simulink model "BLDC_SMO"  (R2024b)
settings: Solver=ode3  StartTime=0.0  StopTime=5  FixedStep=1e-6  RelTol=1e-3
libraries: spsMosfetLib x6, spsCurrentMeasurementLib x3, spsVoltageMeasurementLib x3, simulink x2, spsDCVoltageSourceLib x1, slpidlib x1, spsPermanentMagnetSynchronousMachineLib x1, spspowerguiLib x1
settings Model: Creator=sinha  LastModifiedBy=sinha

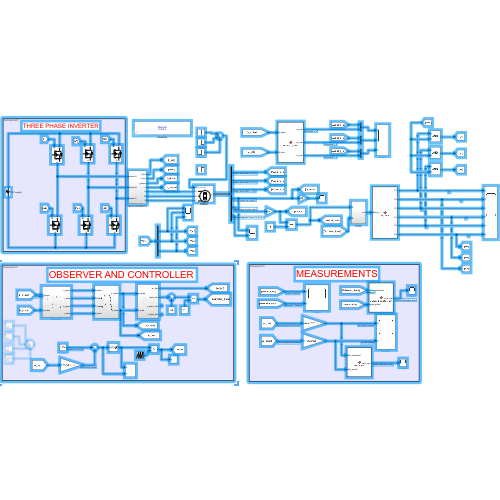
[thumbnail: Simulink's stored preview of the top-level diagram]
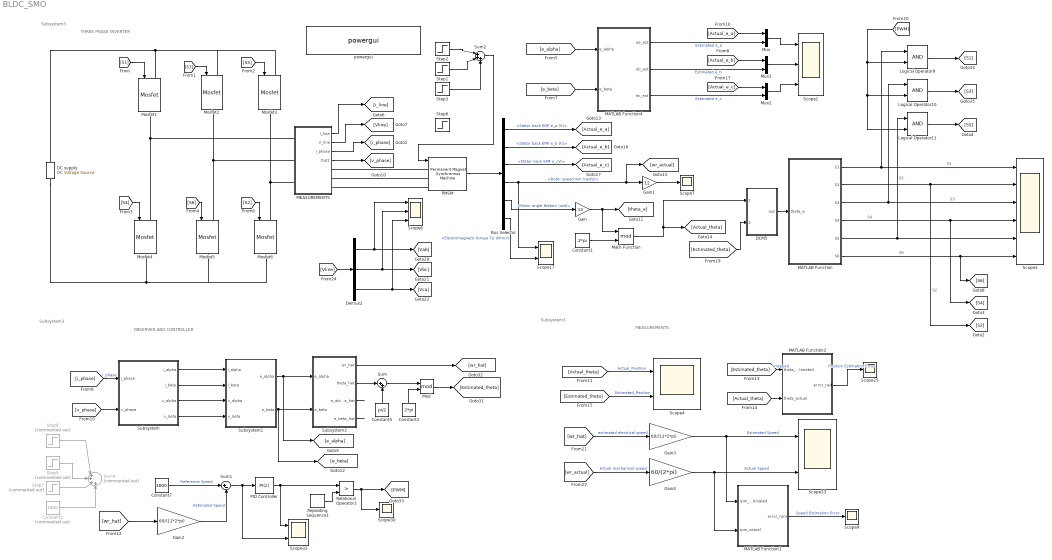
== system BLDC_SMO ==
  note: THREE PHASE INVERTER
  note: Subsystem3
  note: MEASUREMENTS
  note: OBSERVER AND CONTROLLER
  note: Subsystem3
  note: Subsystem3
  Bus Selector : BusSelector  OutputSignals=Stator back EMF e_a (V),Stator back EMF e_b (V),Stator back EMF e_cV),Rotor speed wm (rad/s),Rotor angle thetam (rad),Electromagnetic torque Te (N*m)
  Constant1 : Constant  Value=2*pi
  Constant2 : Constant  Commented=on  Value=1000
  Constant3 : Constant  Value=2*pi
  Constant5 : Constant  Value=pi/2
  Constant7 : Constant  Value=1000
  DC supply : spsDCVoltageSourceLib/DC Voltage Source  Amplitude=120  Measurements=None
  DCM5 : Subsystem
  Demux2 : Demux  Outputs=3
  Gain : Gain  Gain=12
  Gain1 : Gain  Gain=12
  Gain2 : Gain  Gain=60/(12*2*pi)
  Gain3 : Gain  Gain=60/(12*2*pi)
  Gain4 : Gain  Gain=60/(2*pi)
  Logical Operator10 : Logic  AllPortsSameDT=off  OutDataTypeStr=boolean
  Logical Operator11 : Logic  AllPortsSameDT=off  OutDataTypeStr=boolean
  Logical Operator9 : Logic  AllPortsSameDT=off  OutDataTypeStr=boolean
  MATLAB Function : MATLAB Function  TreatAsAtomicUnit=on
  MATLAB Function1 : MATLAB Function  TreatAsAtomicUnit=on  SystemSampleTime=1e-4
  MATLAB Function2 : MATLAB Function  TreatAsAtomicUnit=on  SystemSampleTime=1e-4
  MATLAB Function4 : MATLAB Function  TreatAsAtomicUnit=on  SystemSampleTime=1e-4
  MEASUREMENTS : Subsystem
  Math Function : Math  Operator=mod
  Mod : Math  Operator=mod
  Mosfet{1..6} (6 alike) : spsMosfetLib/Mosfet  Ron=0.1  Lon=0  Rd=0.01  Vfd=0  IC=0  Rs=1e5  Cs=inf  Measurements=off
  Mux : Mux  Inputs=2
  Mux1 : Mux  Inputs=2
  Mux2 : Mux  Inputs=2
  PID Controller : slpidlib/PID Controller  Controller=PI  Form=Parallel  TimeDomain=Discrete-time  UseExternalTs=off  SampleTime=1e-3  IntegratorMethod=Forward Euler  FilterMethod=Forward Euler  ControllerParametersSource=internal  P=0.01  I=0.05  UseKiTs=off  D=0  UseExternalDerivativeSource=off  N=100  UseFilter=on  TunerSelectOption=Transfer Function Based (PID Tuner App)  InitialConditionSource=internal  InitialConditionForIntegrator=0  InitialConditionForFilter=0  DifferentiatorICPrevScaledInput=0  ExternalReset=none  TrackingMode=off  Kt=1  LimitOutput=on  SatLimitsSource=internal  UpperSaturationLimit=1  LowerSaturationLimit=0  LinearizeAsGain=on  AntiWindupMode=back-calculation  Kb=1  LimitIntegrator=off  UpperIntegratorSaturationLimit=inf  LowerIntegratorSaturationLimit=-inf  POutMin=[]  POutMax=[]  IOutMin=[]  IOutMax=[]  DOutMin=[]  DOutMax=[]  NOutMin=[]  NOutMax=[]  SumOutMin=[]  SumOutMax=[]  SaturationOutMin=[]  SaturationOutMax=[]  PParamMin=[]  PParamMax=[]  IParamMin=[]  IParamMax=[]  DParamMin=[]  DParamMax=[]  NParamMin=[]  NParamMax=[]  KbParamMin=[]  KbParamMax=[]  KtParamMin=[]  KtParamMax=[]  KbOutMin=[]  KbOutMax=[]  KtOutMin=[]  KtOutMax=[]  IntegratorOutMin=[]  IntegratorOutMax=[]  FilterOutMin=[]  FilterOutMax=[]  SumI1OutMin=[]  SumI1OutMax=[]  SumI2OutMin=[]  SumI2OutMax=[]  SumI3OutMin=[]  SumI3OutMax=[]  SumI4OutMin=[]  SumI4OutMax=[]  SumDOutMin=[]  SumDOutMax=[]  DifferentiatorOutMin=[]  DifferentiatorOutMax=[]  FilterDiffOutCoefMin=[]  FilterDiffOutCoefMax=[]  ReciprocalOutMin=[]  ReciprocalOutMax=[]  SumDenOutMin=[]  SumDenOutMax=[]  SumNumOutMin=[]  SumNumOutMax=[]  DivideOutMin=[]  DivideOutMax=[]  UdiffTsProdOutMin=[]  UdiffTsProdOutMax=[]  NTsProdOutMin=[]  NTsProdOutMax=[]  UintegralTsProdOutMin=[]  UintegralTsProdOutMax=[]  UngainTsProdOutMin=[]  UngainTsProdOutMax=[]  ClampingZeroOutDataTypeStr=Inherit: Inherit via back propagation  ClampingZeroOutMin=[]  ClampingZeroOutMax=[]  FilterDenConstantOutDataTypeStr=Inherit: Inherit via back propagation  FilterDenConstantOutMin=[]  FilterDenConstantOutMax=[]  PCopyOutDataTypeStr=Inherit: Inherit via back propagation  PCopyOutMin=[]  PCopyOutMax=[]  NCopyOutDataTypeStr=Inherit: Inherit via back propagation  NCopyOutMin=[]  NCopyOutMax=[]  IntegratorContinuousStateAttributes=''  IntegratorStateMustResolveToSignalObject=off  IntegratorRTWStateStorageClass=Auto  FilterContinuousStateAttributes=''  FilterStateMustResolveToSignalObject=off  FilterRTWStateStorageClass=Auto  ParallelPVariant=InternalParameters  IdealPVariant=Disabled  IVariant=InternalParameters  DVariant=Disabled  IntegratorVariant=Discrete  SatVariant=Enabled  AWVariant=BackCalculation  PCopyVariant=Disabled  TRVariant=Disabled  FdbkBlocksVariant=Forward  IdealPFdbkVariant=Disabled  SatFdbkVariant=Disabled  DerivativeFilterVariant=Disabled  NVariant=Disabled  NCopyVariant=Disabled_SignalSpec  FilterICVariant=Disabled  IntegratorICVariant=InternalICs  ExternalResetVariant=Disabled  TRSumVariant=Passthrough  SumFdbkVariant=Disabled  SumVariant=Sum_PI  TsampFilterVariant=InternalTs  TsampNgainVariant=Passthrough  TsampIntegralVariant=Disabled_SignalSpec  ExternalSaturationOutDataTypeStr=Inherit: Same as second input  DerivativeSourceVariant=Disabled  PreIntVariant=InternalPreInt
  PMSM : spsPermanentMagnetSynchronousMachineLib/Permanent Magnet Synchronous Machine  NbPhases=3  FluxDistribution=Trapezoidal  RotorType=Round  MechanicalLoad=Torque Tm  PresetModel=No  ShowDetailedParameters=on  MeasurementBus=off  Resistance=1.5  Inductance=0.5e-3  dqInductances=[8.5e-3, 8.5e-3]  La=0.000835  MachineConstant=Voltage Constant (V_peak L-L / krpm)  Flux=0.027852  VoltageCst=70  TorqueCst=0.66845  Flat=120  Mechanical=[0.008, 1e-3, 12, 0]  PolePairs=4  InitialConditions=[0,0, 0,0]  InitialConditions5ph=[0 0 0 0 0 0]  RefAngle=90 degrees behind phase A axis (modified Park)  IterativeDiscreteModel=Trapezoidal non iterative  TsBlock=-1  TsPowergui=0
  Relational Operator3 : RelationalOperator  Operator=>  OutDataTypeStr=boolean  RndMeth=Simplest  InputSameDT=off
  Repeating Sequence1 : simulink/Sources/Repeating Sequence  rep_seq_t=[0 1e-4]  rep_seq_y=[0 1]
  Scope1 : Scope  NumInputPorts=3
  Scope{4,17,32..33} (4 alike) : Scope  NumInputPorts=2
  Scope{7,9,25,30} (4 alike) : Scope
  Scope3 : Scope  NumInputPorts=6
  Scope6 : Scope  NumInputPorts=3
  Step1 : Step  Time=3  After=-2
  Step2 : Step  Time=2
  Step3 : Step  Time=4
  Step6 : Step  Time=0.99
  Step7 : Step  Commented=on  Time=1.5  After=-50  SampleTime=0
  Step8 : Step  Commented=on  Time=2.5  After=100  SampleTime=0
  Step9 : Step  Commented=on  Time=2  After=-50  SampleTime=0
  Subsystem : Subsystem
  Subsystem1 : Subsystem
  Subsystem2 : Subsystem
  Sum : Sum  Inputs=|++
  Sum1 : Sum  Inputs=|+-
  Sum2 : Sum  Inputs=|+++
  Sum4 : Sum  Commented=on  Inputs=|++++
  powergui : spspowerguiLib/powergui  Priority=2  SimulationMode=Discrete  SampleTime=.000001  frequency=60  Iterations=50  frequencyindice=0  Pbase=100e6  ErrMax=1e-4  UnitsV=kV  UnitsW=MW  buscounter=0  FunctionMessages=off  echomessages=off  EnableUseOfTLC=off  CurrentSourceSwitches=off  DisableSnubberDevices=off  DisableRonSwitches=off  DisableVfSwitches=off  DisplayEquations=off  AutomaticDiscreteSolvers=off  SolverType=Tustin/Backward Euler (TBE)  Interpol=off  ExternalGateDelay=off  methode=off  Ts=0  x0status=blocks  SPID=off  SwTol=0  HookPort=off  NonlinearTolerance=1e-4  nMaxIteration=100  ContinueOnMaxIteration=off  RestoreLinks=warning  ResistiveCurrentMeasurement=off  Frange=[0:2:500]  Ylog=off  Xlog=on  ShowGrid=off  save=off  variable=ZData  structure=0  ZoomFFT=on  StartTime=0.0  cycles=1  DisplayStyle=1  fundamental=60  FreqAxis=off  MaxFrequency=1000  frequencyindicesteady=1  RmsSteady=1  display=off
  wires:
  PMSM/1 -> Bus Selector/1
  Bus Selector/4 -> Gain1/1, [wr_actual], Scope17/1  "<Rotor speed wm (rad/s)>"
  MEASUREMENTS/1(i_line) -> [i_line]
  MEASUREMENTS/2(V_line) -> [Vline]
  Demux2/2 -> Scope6/2, [Vbc]
  [Vline] -> Demux2/1
  Demux2/3 -> Scope6/3, [Vca]
  Demux2/1 -> Scope6/1, [Vab]
  MEASUREMENTS/3(i_phase) -> [i_phase]
  Bus Selector/5 -> Gain/1  "<Rotor angle thetam (rad)>"
  MATLAB Function/1(S1) -> Logical Operator9/1, Scope3/1  "S1"
  MATLAB Function/2(S2) -> Scope3/2, [S2]  "S2"
  MATLAB Function/6(S6) -> Scope3/6, [S6]  "S6"
  MATLAB Function/4(S4) -> Scope3/4, [S4]  "S4"
  MATLAB Function/3(S3) -> Logical Operator10/1, Scope3/3  "S3"
  MATLAB Function/5(S5) -> Logical Operator11/1, Scope3/5  "S5"
  MEASUREMENTS/4(Out1) -> [v_phase]
  Gain/1 -> [theta_e], Math Function/1
  Constant1/1 -> Math Function/2
  Math Function/1 -> DCM5/1(1), [Actual_theta]
  Gain1/1 -> Scope7/1
  Bus Selector/6 -> Scope17/2  "<Electromagnetic torque Te (N*m)>"
  [Estimated_theta] -> DCM5/2(2)
  [PWM] -> Logical Operator11/2, Logical Operator10/2, Logical Operator9/2
  Logical Operator9/1 -> [S1]
  Logical Operator10/1 -> [S3]
  Logical Operator11/1 -> [S5]
  DCM5/1(out) -> MATLAB Function/1(theta_e)
  Step2/1 -> Sum2/1
  Step1/1 -> Sum2/2
  Step3/1 -> Sum2/3
  MATLAB Function4/1(ea_est) -> Mux/2  "Estimated e_a"
  MATLAB Function4/2(eb_est) -> Mux1/2  "Estimated e_b"
  MATLAB Function4/3(ec_est) -> Mux2/2  "Estimated e_c"
  Mux/1 -> Scope1/1
  Mux1/1 -> Scope1/2
  Mux2/1 -> Scope1/3
  [e_alpha] -> MATLAB Function4/1(e_alpha)
  [e_beta] -> MATLAB Function4/2(e_beta)
  Bus Selector/1 -> [Actual_e_a]  "<Stator back EMF e_a (V)>"
  Bus Selector/3 -> [Actual_e_c]  "<Stator back EMF e_cV)>"
  Bus Selector/2 -> [Actual_e_b]  "<Stator back EMF e_b (V)>"
  [Actual_e_b] -> Mux1/1
  [Actual_e_a] -> Mux/1
  [Actual_e_c] -> Mux2/1
  MATLAB Function1/1(error_rpm) -> Scope9/1  "Speed Estimation Error"
  [Estimated_theta] -> Scope4/2  "Estimated_Position"
  Gain3/1 -> MATLAB Function1/1(rpm_estimated), Scope33/1  "Estimated Speed"
  MATLAB Function2/1(error_rad) -> Scope25/1  "Position Estimation Error"
  [wr_hat] -> Gain3/1  "estimated electrical speed"
  [Actual_theta] -> Scope4/1  "Actual_Position"
  [wr_actual] -> Gain4/1  "Actual mechanical speed"
  Gain4/1 -> MATLAB Function1/2(rpm_actual), Scope33/2  "Actual Spped"
  [Actual_theta] -> MATLAB Function2/2(theta_actual)
  [Estimated_theta] -> MATLAB Function2/1(theta_estimated)  "wrapped"
  Subsystem2/4(e_beta_hat) -> ?
  Subsystem2/2(theta_hat) -> Sum/1
  Sum1/1 -> PID Controller/1, Scope32/2
  Sum/1 -> Mod/1
  Repeating Sequence1/1 -> Relational Operator3/2
  Step8/1 -> Sum4/1
  Subsystem2/3(e_alpha_hat) -> ?
  PID Controller/1 -> Scope32/1, Relational Operator3/1
  Constant5/1 -> Sum/2
  Relational Operator3/1 -> [PWM], Scope30/1
  [i_phase] -> Subsystem/1(i_phase)  "i_phase"
  Mod/1 -> [Estimated_theta]
  [wr_hat] -> Gain2/1
  Subsystem/1(i_alpha) -> Subsystem1/1(i_alpha)
  Subsystem2/1(wr_hat) -> [wr_hat]
  [v_phase] -> Subsystem/2(v_phase)
  Constant3/1 -> Mod/2
  Subsystem/2(i_beta) -> Subsystem1/2(i_beta)
  Constant2/1 -> Sum4/4
  Subsystem/3(v_alpha) -> Subsystem1/3(v_alpha)
  Subsystem1/2(e_beta) -> [e_beta], Subsystem2/2(e_beta)
  Gain2/1 -> Sum1/2  "Estimated Speed"
  Step7/1 -> Sum4/3
  Subsystem/4(v_beta) -> Subsystem1/4(v_beta)
  Subsystem1/1(e_alpha) -> Subsystem2/1(e_alpha), [e_alpha]
  Step9/1 -> Sum4/2
  [S6] -> Mosfet5/1
  [S3] -> Mosfet2/1
  [S1] -> Mosfet1/1
  [S2] -> Mosfet6/1
  [S4] -> Mosfet4/1
  [S5] -> Mosfet3/1
  Constant7/1 -> Sum1/1  "Reference Speed"
  Sum2/1 -> PMSM/1
  connections:
  PMSM/LConn1 -- MEASUREMENTS/RConn1
  PMSM/LConn2 -- MEASUREMENTS/RConn2
  PMSM/LConn3 -- MEASUREMENTS/RConn3
  Mosfet6/LConn1 -- Mosfet3/RConn1 -- MEASUREMENTS/LConn3
  DC supply/LConn1 -- Mosfet6/RConn1 -- Mosfet5/RConn1 -- Mosfet4/RConn1
  Mosfet5/LConn1 -- MEASUREMENTS/LConn2 -- Mosfet2/RConn1
  Mosfet3/LConn1 -- Mosfet2/LConn1 -- Mosfet1/LConn1 -- DC supply/RConn1
  Mosfet4/LConn1 -- MEASUREMENTS/LConn1 -- Mosfet1/RConn1

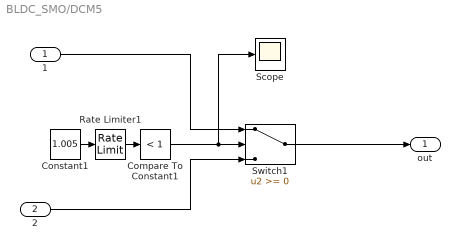
== system BLDC_SMO/DCM5 ==
  1 : Inport
  2 : Inport  Port=2
  Compare To Constant1 : simulink/Logic and Bit Operations/Compare To Constant  relop=<  const=1  OutDataTypeStr=boolean
  Constant1 : Constant  Value=1.005  OutDataTypeStr=double  SampleTime=1/5000
  Rate Limiter1 : RateLimiter  RisingSlewLimit=1/0.2  FallingSlewLimit=0  SampleTimeMode=inherited
  Scope : Scope
  Switch1 : Switch  OutMin=[-230]  OutMax=[230]  OutDataTypeStr=double  SaturateOnIntegerOverflow=off  InputSameDT=off
  out : Outport  VectorParamsAs1DForOutWhenUnconnected=off
  wires:
  1/1 -> Switch1/1
  2/1 -> Switch1/3
  Switch1/1 -> out/1
  Constant1/1 -> Rate Limiter1/1
  Rate Limiter1/1 -> Compare To Constant1/1
  Compare To Constant1/1 -> Switch1/2, Scope/1

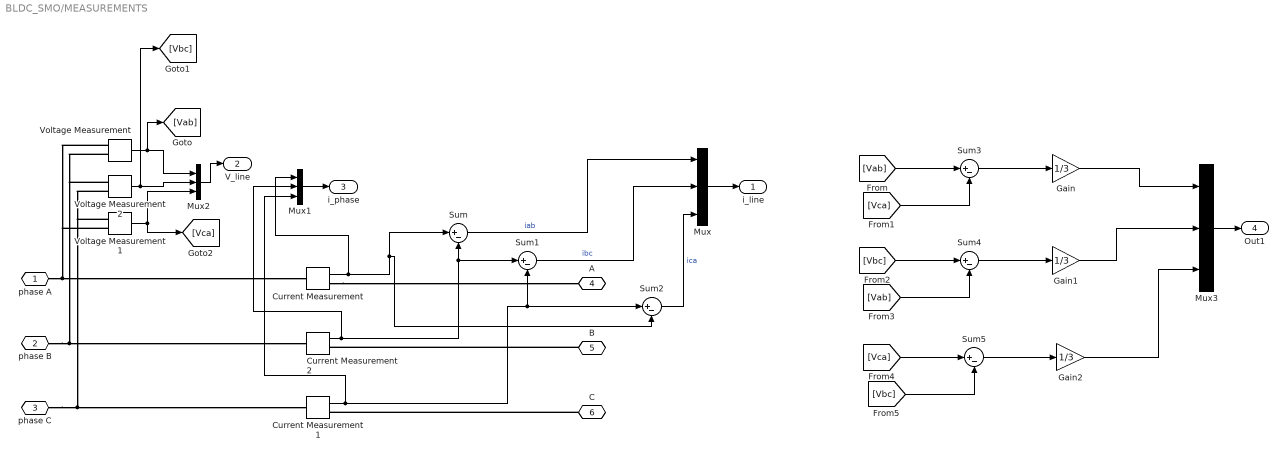
== system BLDC_SMO/MEASUREMENTS ==
  Current Measurement : spsCurrentMeasurementLib/Current Measurement  PhasorSimulation=off  OutputType=Complex  PSBequivalent=0
  Current Measurement1 : spsCurrentMeasurementLib/Current Measurement  PhasorSimulation=off  OutputType=Complex  PSBequivalent=0
  Current Measurement2 : spsCurrentMeasurementLib/Current Measurement  PhasorSimulation=off  OutputType=Complex  PSBequivalent=0
  Gain : Gain  Gain=1/3
  Gain1 : Gain  Gain=1/3
  Gain2 : Gain  Gain=1/3
  Mux{,1..3} (4 alike) : Mux  Inputs=3
  Sum{,1..5} (6 alike) : Sum  Inputs=|+-
  Voltage Measurement : spsVoltageMeasurementLib/Voltage Measurement  PhasorSimulation=off  OutputType=Complex  PSBequivalent=0
  Voltage Measurement1 : spsVoltageMeasurementLib/Voltage Measurement  PhasorSimulation=off  OutputType=Complex  PSBequivalent=0
  Voltage Measurement2 : spsVoltageMeasurementLib/Voltage Measurement  PhasorSimulation=off  OutputType=Complex  PSBequivalent=0
  phase A : PMIOPort  Side=Left
  phase B : PMIOPort  Port=2  Side=Left
  phase C : PMIOPort  Port=3  Side=Left
  A : PMIOPort  Port=4  Side=Right
  B : PMIOPort  Port=5  Side=Right
  C : PMIOPort  Port=6  Side=Right
  i_line : Outport
  V_line : Outport  Port=2
  i_phase : Outport  Port=3
  Out1 : Outport  Port=4
  wires:
  Current Measurement/1 -> Mux1/1, Sum2/2, Sum/1
  Current Measurement2/1 -> Mux1/2, Sum1/1, Sum/2
  Sum/1 -> Mux/1  "iab"
  Current Measurement1/1 -> Mux1/3, Sum2/1, Sum1/2
  Sum1/1 -> Mux/2  "ibc"
  Sum2/1 -> Mux/3  "ica"
  Mux/1 -> i_line/1
  Mux1/1 -> i_phase/1
  Voltage Measurement/1 -> Mux2/1, [Vab]
  Voltage Measurement2/1 -> [Vbc], Mux2/2
  Voltage Measurement1/1 -> [Vca], Mux2/3
  Mux2/1 -> V_line/1
  [Vca] -> Sum3/2
  [Vab] -> Sum3/1
  Sum3/1 -> Gain/1
  Sum4/1 -> Gain1/1
  [Vab] -> Sum4/2
  [Vbc] -> Sum4/1
  Sum5/1 -> Gain2/1
  [Vbc] -> Sum5/2
  [Vca] -> Sum5/1
  Gain/1 -> Mux3/1
  Gain1/1 -> Mux3/2
  Gain2/1 -> Mux3/3
  Mux3/1 -> Out1/1
  connections:
  phase A/RConn1 -- Voltage Measurement1/LConn2 -- Voltage Measurement/LConn1 -- Current Measurement/LConn1
  Current Measurement/RConn1 -- A/RConn1
  phase B/RConn1 -- Voltage Measurement2/LConn1 -- Voltage Measurement/LConn2 -- Current Measurement2/LConn1
  phase C/RConn1 -- Voltage Measurement1/LConn1 -- Voltage Measurement2/LConn2 -- Current Measurement1/LConn1
  B/RConn1 -- Current Measurement2/RConn1
  C/RConn1 -- Current Measurement1/RConn1

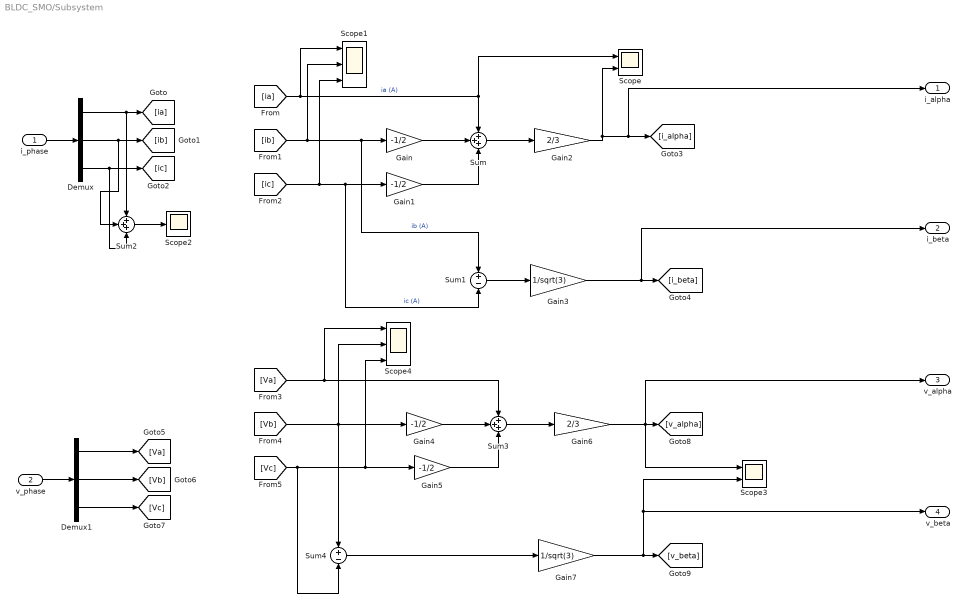
== system BLDC_SMO/Subsystem ==
  i_phase : Inport
  v_phase : Inport  Port=2
  Demux : Demux  Outputs=3
  Demux1 : Demux  Outputs=3
  Gain{,1,4..5} (4 alike) : Gain  Gain=-1/2
  Gain2 : Gain  Gain=2/3
  Gain3 : Gain  Gain=1/sqrt(3)
  Gain6 : Gain  Gain=2/3
  Gain7 : Gain  Gain=1/sqrt(3)
  Scope : Scope  NumInputPorts=2
  Scope1 : Scope  NumInputPorts=3
  Scope2 : Scope
  Scope3 : Scope  NumInputPorts=2
  Scope4 : Scope  NumInputPorts=3
  Sum : Sum  Inputs=+++
  Sum1 : Sum  Inputs=+-
  Sum2 : Sum  Inputs=+++
  Sum3 : Sum  Inputs=+++
  Sum4 : Sum  Inputs=+-
  i_alpha : Outport
  i_beta : Outport  Port=2
  v_alpha : Outport  Port=3
  v_beta : Outport  Port=4
  wires:
  i_phase/1 -> Demux/1
  Demux/1 -> Sum2/1, [ia]
  Demux/3 -> Sum2/3, [ic]
  Demux/2 -> Sum2/2, [ib]
  [ia] -> Scope1/1, Scope/1, Sum/1  "ia (A)"
  [ib] -> Scope1/2, Sum1/1, Gain/1  "ib (A)"
  [ic] -> Scope1/3, Sum1/2, Gain1/1  "ic (A)"
  Gain1/1 -> Sum/3
  Gain/1 -> Sum/2
  Sum/1 -> Gain2/1
  Sum1/1 -> Gain3/1
  Gain2/1 -> Scope/2, i_alpha/1, [i_alpha]
  Gain3/1 -> i_beta/1, [i_beta]
  Sum2/1 -> Scope2/1
  v_phase/1 -> Demux1/1
  Demux1/1 -> [Va]
  Demux1/2 -> [Vb]
  Demux1/3 -> [Vc]
  [Va] -> Scope4/1, Sum3/1
  [Vb] -> Scope4/2, Gain4/1, Sum4/1
  Gain4/1 -> Sum3/2
  Gain5/1 -> Sum3/3
  [Vc] -> Sum4/2, Scope4/3, Gain5/1
  Sum3/1 -> Gain6/1
  Sum4/1 -> Gain7/1
  Gain7/1 -> v_beta/1, Scope3/2, [v_beta]
  Gain6/1 -> Scope3/1, v_alpha/1, [v_alpha]

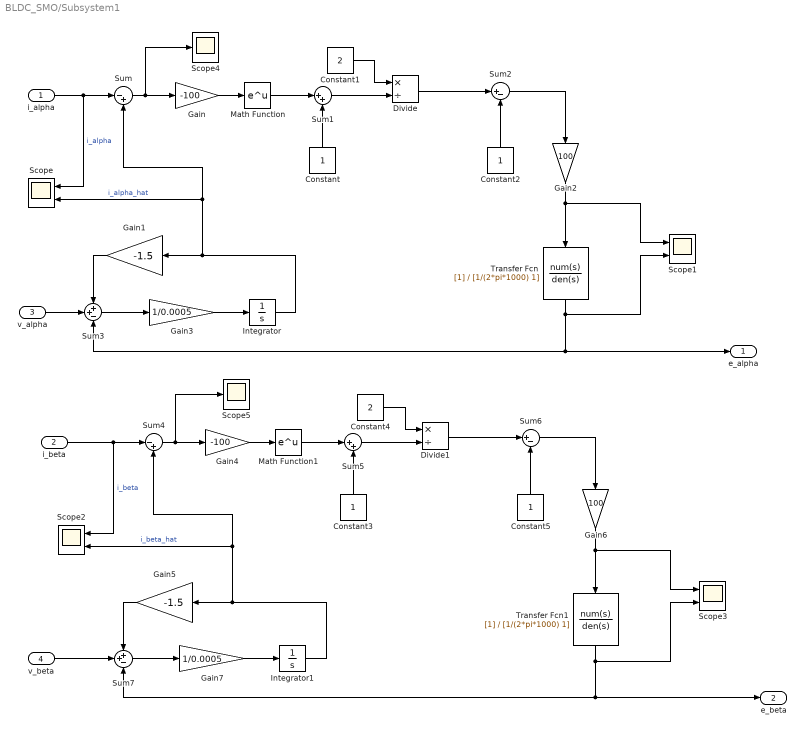
== system BLDC_SMO/Subsystem1 ==
  i_alpha : Inport
  i_beta : Inport  Port=2
  v_alpha : Inport  Port=3
  v_beta : Inport  Port=4
  Constant{,2..3,5} (4 alike) : Constant
  Constant1 : Constant  Value=2
  Constant4 : Constant  Value=2
  Divide : Product  Inputs=*/
  Divide1 : Product  Inputs=*/
  Gain : Gain  Gain=-100
  Gain1 : Gain  Gain=-1.5
  Gain2 : Gain  Gain=100
  Gain3 : Gain  Gain=1/0.0005
  Gain4 : Gain  Gain=-100
  Gain5 : Gain  Gain=-1.5
  Gain6 : Gain  Gain=100
  Gain7 : Gain  Gain=1/0.0005
  Integrator : Integrator
  Integrator1 : Integrator
  Math Function : Math
  Math Function1 : Math
  Scope{,1..3} (4 alike) : Scope  NumInputPorts=2
  Scope4 : Scope
  Scope5 : Scope
  Sum : Sum  Inputs=|-+
  Sum1 : Sum  Inputs=|++
  Sum2 : Sum  Inputs=|+-
  Sum3 : Sum  Inputs=++-
  Sum4 : Sum  Inputs=|-+
  Sum5 : Sum  Inputs=|++
  Sum6 : Sum  Inputs=|+-
  Sum7 : Sum  Inputs=++-
  Transfer Fcn : TransferFcn  Denominator=[1/(2*pi*1000) 1]
  Transfer Fcn1 : TransferFcn  Denominator=[1/(2*pi*1000) 1]
  e_alpha : Outport
  e_beta : Outport  Port=2
  wires:
  i_alpha/1 -> Scope/1, Sum/1  "i_alpha"
  Gain/1 -> Math Function/1
  Constant/1 -> Sum1/2
  Math Function/1 -> Sum1/1
  Sum1/1 -> Divide/2
  Constant1/1 -> Divide/1
  Divide/1 -> Sum2/1
  Constant2/1 -> Sum2/2
  v_alpha/1 -> Sum3/2
  Sum2/1 -> Gain2/1
  Sum3/1 -> Gain3/1
  Gain3/1 -> Integrator/1
  Integrator/1 -> Sum/2, Scope/2, Gain1/1  "i_alpha_hat"
  Gain1/1 -> Sum3/1
  Gain2/1 -> Scope1/1, Transfer Fcn/1
  Sum/1 -> Scope4/1, Gain/1
  Transfer Fcn/1 -> Scope1/2, Sum3/3, e_alpha/1
  Transfer Fcn1/1 -> e_beta/1, Sum7/3, Scope3/2
  Sum4/1 -> Gain4/1, Scope5/1
  Gain6/1 -> Transfer Fcn1/1, Scope3/1
  Gain5/1 -> Sum7/1
  Integrator1/1 -> Gain5/1, Scope2/2, Sum4/2  "i_beta_hat"
  Gain7/1 -> Integrator1/1
  Sum7/1 -> Gain7/1
  Sum6/1 -> Gain6/1
  v_beta/1 -> Sum7/2
  Constant5/1 -> Sum6/2
  Divide1/1 -> Sum6/1
  Constant4/1 -> Divide1/1
  Sum5/1 -> Divide1/2
  Math Function1/1 -> Sum5/1
  Constant3/1 -> Sum5/2
  Gain4/1 -> Math Function1/1
  i_beta/1 -> Sum4/1, Scope2/1  "i_beta"

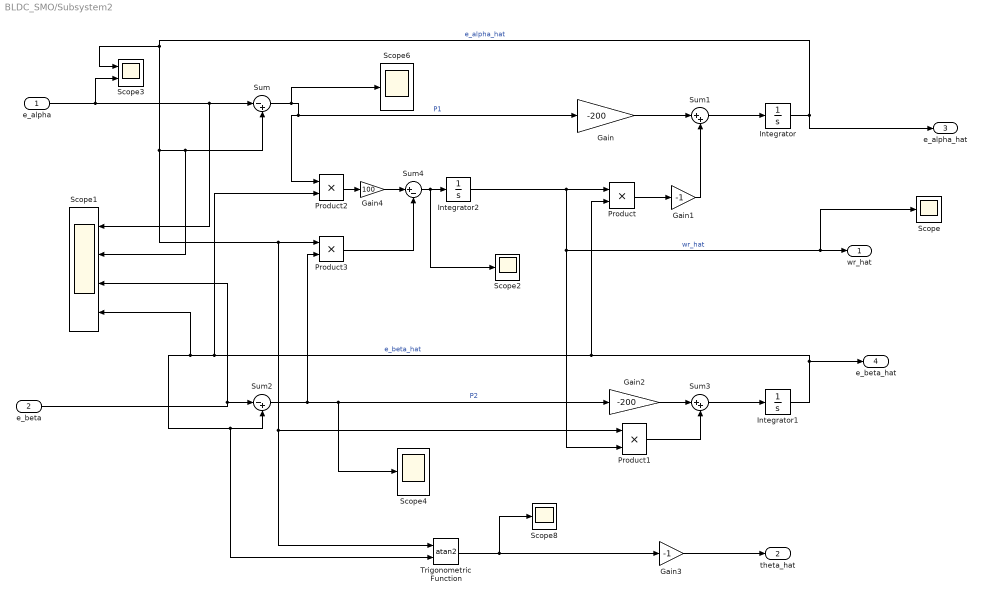
== system BLDC_SMO/Subsystem2 ==
  e_alpha : Inport
  e_beta : Inport  Port=2
  Gain : Gain  Gain=-200
  Gain1 : Gain  Gain=-1
  Gain2 : Gain  Gain=-200
  Gain3 : Gain  Gain=-1
  Gain4 : Gain  Gain=100
  Integrator : Integrator
  Integrator1 : Integrator
  Integrator2 : Integrator
  Product{,1..3} (4 alike) : Product
  Scope{,2,4,6,8} (5 alike) : Scope
  Scope1 : Scope  NumInputPorts=4
  Scope3 : Scope  NumInputPorts=2
  Sum : Sum  Inputs=|-+
  Sum1 : Sum  Inputs=|++
  Sum2 : Sum  Inputs=|-+
  Sum3 : Sum  Inputs=|++
  Sum4 : Sum  Inputs=|+-
  Trigonometric Function : Trigonometry  Operator=atan2
  wr_hat : Outport
  theta_hat : Outport  Port=2
  e_alpha_hat : Outport  Port=3
  e_beta_hat : Outport  Port=4
  wires:
  Product/1 -> Gain1/1
  Gain/1 -> Sum1/1
  Sum1/1 -> Integrator/1
  Integrator/1 -> Scope3/1, Scope1/2, Sum/2, Product1/1, Trigonometric Function/1, Product3/1, e_alpha_hat/1  "e_alpha_hat"
  Integrator1/1 -> e_beta_hat/1, Product2/2, Scope1/4, Trigonometric Function/2, Sum2/2, Product/2  "e_beta_hat"
  Sum3/1 -> Integrator1/1
  Gain2/1 -> Sum3/1
  Sum2/1 -> Product3/2, Scope4/1, Gain2/1  "P2"
  Product2/1 -> Gain4/1
  Product3/1 -> Sum4/2
  Integrator2/1 -> Product1/2, Scope/1, wr_hat/1, Product/1  "wr_hat"
  e_alpha/1 -> Scope3/2, Sum/1, Scope1/1
  e_beta/1 -> Scope1/3, Sum2/1
  Sum/1 -> Scope6/1, Product2/1, Gain/1  "P1"
  Sum4/1 -> Scope2/1, Integrator2/1
  Gain1/1 -> Sum1/2
  Product1/1 -> Sum3/2
  Trigonometric Function/1 -> Scope8/1, Gain3/1
  Gain3/1 -> theta_hat/1
  Gain4/1 -> Sum4/1

== matlab function BLDC_SMO/MATLAB Function1 ==
  data: rpm_estimated input; rpm_actual input; error_rpm output
function error_rpm = rpm_error(rpm_estimated, rpm_actual)

error_rpm = rpm_estimated - rpm_actual;

end

== matlab function BLDC_SMO/MATLAB Function ==
  data: theta_e input; S1 output; S2 output; S3 output; S4 output; S5 output; S6 output
function [S1,S2,S3,S4,S5,S6] = six_step(theta_e)

theta_e = mod(theta_e, 2*pi);
% 60-degree sector
sector = floor(theta_e/(pi/3)) + 1;

% Default: all switches OFF
S1 = 0;
S2 = 0;
S3 = 0;
S4 = 0;
S5 = 0;
S6 = 0;

switch sector

    case 1
        % A+ B-
        S1 = 1;
        S6 = 1;

    case 2
        % A+ C-
        S1 = 1;
        S2 = 1;

    case 3
        % B+ C-
        S3 = 1;
        S2 = 1;

    case 4
        % B+ A-
        S3 = 1;
        S4 = 1;

    case 5
        % C+ A-
        S5 = 1;
        S4 = 1;

    case 6
        % C+ B-
        S5 = 1;
        S6 = 1;

end

== matlab function BLDC_SMO/MATLAB Function2 ==
  data: theta_estimated input; theta_actual input; error_rad output

function error_rad = wrapped_angle_error(theta_estimated, theta_actual)

delta_theta = theta_estimated - theta_actual;

error_rad = atan2(sin(delta_theta), cos(delta_theta));

end

== matlab function BLDC_SMO/MATLAB Function4 ==
  data: e_alpha input; e_beta input; ea_est output; eb_est output; ec_est output

function [ea_est, eb_est, ec_est] = inverse_clarke(e_alpha, e_beta)

ea_est = e_alpha;

eb_est = -0.5*e_alpha + (sqrt(3)/2)*e_beta;

ec_est = -0.5*e_alpha - (sqrt(3)/2)*e_beta;

end
